simulink model "IntegratedFormationOptical"  (R2026a)
settings: Solver=ode4  StopTime=Tend  FixedStep=Ts
model workspace (MAT data in the model file):
  CASE = 3
  MODE = 2
  TACQ = 40
  TAUCPA = 0.005
  TX = [1; 1; 1; 2; 3]
  Tend = 50
  Ts = 0.001
  c0 = [0.824168944005; -0.579250814418; 0.824168944005; -0.579250814418; 0.824168944005; -0.579250814418; 0.676400226361; -0.507300169771; 0.44019405004; 0.711385027297]
  cfg.n = 4
  cfg.topology = 'mesh'
  cfg.seed = 101
  cfg.dt = 0.02
  cfg.T = 50
  cfg.J = 0.002
  cfg.b = 0.004
  cfg.tau = 0.08
  cfg.umax = 2e-06
  cfg.rateMax = 0.00012
  cfg.lambda = 8
  cfg.K = 8e-05
  cfg.phi = 8e-06
  cfg.kp = 64
  cfg.kd = 14
  cfg.ki = 8
  cfg.initialAngle = [2e-06; -1e-06]
  cfg.noise = 8e-08
  cfg.powerNoise = 0.008
  cfg.Pt = 0.5
  cfg.eta = 0.4
  cfg.divergence = 2e-05
  cfg.aperture = 0.1
  cfg.distance = 800000
  cfg.sensitivity = 1.5e-06
  cfg.capacity = 1000000000
  cfg.offered = 600000000
  cfg.packetBits = 12000
  cfg.c = 299792458
  cfg.processing = 0.0001
  cfg.method = 'proposed'
  cfg.controller = 'SMC'
  cfg.scenario = 'normal'
  cfg.faultStart = 42
  cfg.faultEnd = 48
  cfg.profile = 'sudden'
  cfg.severity = 1
  cfg.probeAmplitude = 6e-06
  cfg.probeDwell = 0.5
  cfg.maxCorrection = 3.5e-05
  cfg.detectRatio = 0.72
  cfg.decisionPeriod = 0.1
  cfg.warmup = 41
  cfg.edges = [1  2; 1  3; 1  4; 2  3; 3  4]
  cfg.m = 5
  cfg.version = '1.0.0'
  cfg.assumptions = 'Fixed sparse graph; one effective two-axis terminal per bidirectional edge; fluid single flow 1 to 2; no orbital propagation or atmospheric loss.'
  cfg.noiseSamples = [0.0535121228343 0.398971857605 -3.13116194418 0.785317147926 -0.646255228153 0.891855797063 0.932023533057 -1.5355153092 0.0745919923426 -0.661062844199 -0.294971205653 0.972557875124 ... (62625 elements, 2505x5x5)]
  distData = [0  0  0  0  0  0  0  0  0  0  0  0  0; 1  0  0  0  0  0  0  0  0  0  0  0  0; 2  0  0  0  0  0  0  0  0  0  0  0  0; 51  0  0  0  0  0  0  0  0  0  0  0  0]
  umax = 0.2
  x0 = [0.15; 0.22; -0.15; 0.15; -0.08; 0.12; 0.08; 0.18; -0.13; -0.14; 0.11; 0.13; -0.09; 0.12; 0.18; 0.16; 0.12; -0.07; 0.12; -0.13; 0.15; -0.13; -0.17; 0.12]
undefined symbols (not defined in the file or in its folder): terminal_parameters
settings Model: Creator=kaush  LastModifiedBy=kaush

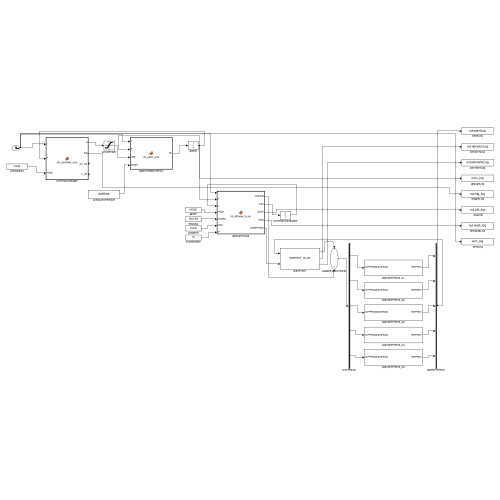
[thumbnail: Simulink's stored preview of the top-level diagram]
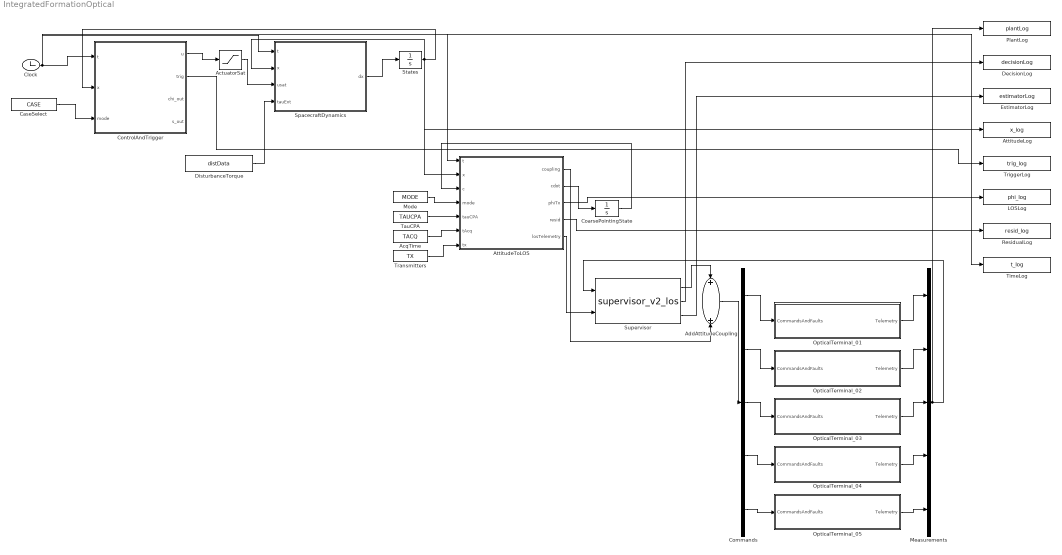
== system IntegratedFormationOptical ==
  AcqTime : Constant  Value=TACQ
  ActuatorSat : Saturate  UpperLimit=umax  LowerLimit=-umax
  AddAttitudeCoupling : Sum
  AttitudeLog : ToWorkspace  VariableName=x_log  SampleTime=cfg.dt
  AttitudeToLOS : MATLAB Function  TreatAsAtomicUnit=on
  CaseSelect : Constant  Value=CASE
  Clock : Clock
  CoarsePointingState : Integrator  InitialCondition=c0
  Commands : Demux  Outputs=[11 11 11 11 11]
  ControlAndTrigger : MATLAB Function  TreatAsAtomicUnit=on
  DecisionLog : ToWorkspace  VariableName=decisionLog  SaveFormat=Timeseries  SampleTime=-1
  DisturbanceTorque : FromWorkspace  VariableName=distData  Interpolate=off  OutputAfterFinalValue=Holding final value
  EstimatorLog : ToWorkspace  VariableName=estimatorLog  SaveFormat=Timeseries  SampleTime=-1
  LOSLog : ToWorkspace  VariableName=phi_log  SampleTime=cfg.dt
  Measurements : Mux  Inputs=5
  Mode : Constant  Value=MODE
  OpticalTerminal_01 : Subsystem
  OpticalTerminal_02 : Subsystem
  OpticalTerminal_03 : Subsystem
  OpticalTerminal_04 : Subsystem
  OpticalTerminal_05 : Subsystem
  PlantLog : ToWorkspace  VariableName=plantLog  SaveFormat=Timeseries  SampleTime=cfg.dt
  ResidualLog : ToWorkspace  VariableName=resid_log  SampleTime=cfg.dt
  SpacecraftDynamics : MATLAB Function  TreatAsAtomicUnit=on
  States : Integrator  InitialCondition=x0
  Supervisor : M-S-Function  FunctionName=supervisor_v2_los  Parameters=cfg
  TauCPA : Constant  Value=TAUCPA
  TimeLog : ToWorkspace  VariableName=t_log  SampleTime=cfg.dt
  Transmitters : Constant  Value=TX
  TriggerLog : ToWorkspace  VariableName=trig_log  SampleTime=Ts
  wires:
  Clock/1 -> ControlAndTrigger/1(t), SpacecraftDynamics/1(t), AttitudeToLOS/1(t), TimeLog/1
  States/1 -> ControlAndTrigger/2(x), SpacecraftDynamics/2(x), AttitudeToLOS/2(x), AttitudeLog/1
  CaseSelect/1 -> ControlAndTrigger/3(mode)
  ControlAndTrigger/1(u) -> ActuatorSat/1
  ActuatorSat/1 -> SpacecraftDynamics/3(usat)
  DisturbanceTorque/1 -> SpacecraftDynamics/4(tauExt)
  SpacecraftDynamics/1(dx) -> States/1
  CoarsePointingState/1 -> AttitudeToLOS/3(c)
  Mode/1 -> AttitudeToLOS/4(mode)
  TauCPA/1 -> AttitudeToLOS/5(tauCPA)
  AcqTime/1 -> AttitudeToLOS/6(tAcq)
  Transmitters/1 -> AttitudeToLOS/7(tx)
  AttitudeToLOS/2(cdot) -> CoarsePointingState/1
  Supervisor/1 -> AddAttitudeCoupling/1
  AttitudeToLOS/1(coupling) -> AddAttitudeCoupling/2
  AddAttitudeCoupling/1 -> Commands/1
  Commands/1 -> OpticalTerminal_01/1(CommandsAndFaults)
  OpticalTerminal_01/1(Telemetry) -> Measurements/1
  Commands/2 -> OpticalTerminal_02/1(CommandsAndFaults)
  OpticalTerminal_02/1(Telemetry) -> Measurements/2
  Commands/3 -> OpticalTerminal_03/1(CommandsAndFaults)
  OpticalTerminal_03/1(Telemetry) -> Measurements/3
  Commands/4 -> OpticalTerminal_04/1(CommandsAndFaults)
  OpticalTerminal_04/1(Telemetry) -> Measurements/4
  Commands/5 -> OpticalTerminal_05/1(CommandsAndFaults)
  OpticalTerminal_05/1(Telemetry) -> Measurements/5
  Measurements/1 -> Supervisor/1, PlantLog/1
  AttitudeToLOS/5(losTelemetry) -> Supervisor/2
  Supervisor/2 -> DecisionLog/1
  Supervisor/3 -> EstimatorLog/1
  ControlAndTrigger/2(trig) -> TriggerLog/1
  AttitudeToLOS/3(phiTx) -> LOSLog/1
  AttitudeToLOS/4(resid) -> ResidualLog/1

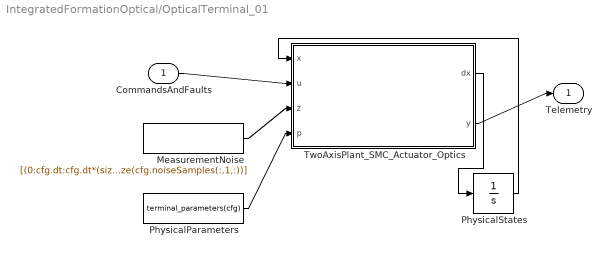
== system IntegratedFormationOptical/OpticalTerminal_01 ==
  CommandsAndFaults : Inport
  MeasurementNoise : FromWorkspace  VariableName=[(0:cfg.dt:cfg.dt*(size(cfg.noiseSamples,1)-1))' squeeze(cfg.noiseSamples(:,1,:))]  Interpolate=off  OutputAfterFinalValue=Holding final value
  PhysicalParameters : Constant  Value=terminal_parameters(cfg)
  PhysicalStates : Integrator  InitialCondition=[cfg.initialAngle;zeros(6,1)]
  TwoAxisPlant_SMC_Actuator_Optics : MATLAB Function  TreatAsAtomicUnit=on
  Telemetry : Outport
  wires:
  CommandsAndFaults/1 -> TwoAxisPlant_SMC_Actuator_Optics/2(u)
  PhysicalStates/1 -> TwoAxisPlant_SMC_Actuator_Optics/1(x)
  MeasurementNoise/1 -> TwoAxisPlant_SMC_Actuator_Optics/3(z)
  PhysicalParameters/1 -> TwoAxisPlant_SMC_Actuator_Optics/4(p)
  TwoAxisPlant_SMC_Actuator_Optics/1(dx) -> PhysicalStates/1
  TwoAxisPlant_SMC_Actuator_Optics/2(y) -> Telemetry/1

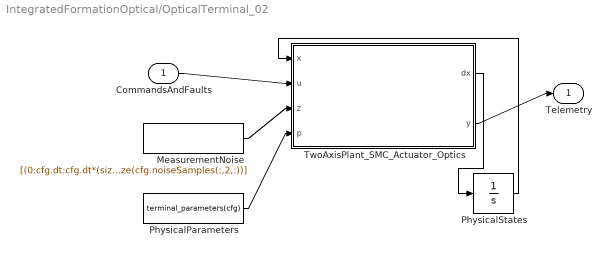
== system IntegratedFormationOptical/OpticalTerminal_02 ==
  CommandsAndFaults : Inport
  MeasurementNoise : FromWorkspace  VariableName=[(0:cfg.dt:cfg.dt*(size(cfg.noiseSamples,1)-1))' squeeze(cfg.noiseSamples(:,2,:))]  Interpolate=off  OutputAfterFinalValue=Holding final value
  PhysicalParameters : Constant  Value=terminal_parameters(cfg)
  PhysicalStates : Integrator  InitialCondition=[cfg.initialAngle;zeros(6,1)]
  TwoAxisPlant_SMC_Actuator_Optics : MATLAB Function  TreatAsAtomicUnit=on
  Telemetry : Outport
  wires:
  CommandsAndFaults/1 -> TwoAxisPlant_SMC_Actuator_Optics/2(u)
  PhysicalStates/1 -> TwoAxisPlant_SMC_Actuator_Optics/1(x)
  MeasurementNoise/1 -> TwoAxisPlant_SMC_Actuator_Optics/3(z)
  PhysicalParameters/1 -> TwoAxisPlant_SMC_Actuator_Optics/4(p)
  TwoAxisPlant_SMC_Actuator_Optics/1(dx) -> PhysicalStates/1
  TwoAxisPlant_SMC_Actuator_Optics/2(y) -> Telemetry/1

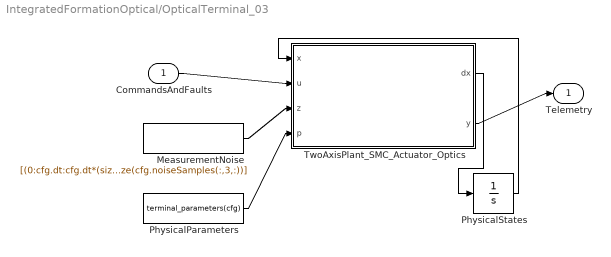
== system IntegratedFormationOptical/OpticalTerminal_03 ==
  CommandsAndFaults : Inport
  MeasurementNoise : FromWorkspace  VariableName=[(0:cfg.dt:cfg.dt*(size(cfg.noiseSamples,1)-1))' squeeze(cfg.noiseSamples(:,3,:))]  Interpolate=off  OutputAfterFinalValue=Holding final value
  PhysicalParameters : Constant  Value=terminal_parameters(cfg)
  PhysicalStates : Integrator  InitialCondition=[cfg.initialAngle;zeros(6,1)]
  TwoAxisPlant_SMC_Actuator_Optics : MATLAB Function  TreatAsAtomicUnit=on
  Telemetry : Outport
  wires:
  CommandsAndFaults/1 -> TwoAxisPlant_SMC_Actuator_Optics/2(u)
  PhysicalStates/1 -> TwoAxisPlant_SMC_Actuator_Optics/1(x)
  MeasurementNoise/1 -> TwoAxisPlant_SMC_Actuator_Optics/3(z)
  PhysicalParameters/1 -> TwoAxisPlant_SMC_Actuator_Optics/4(p)
  TwoAxisPlant_SMC_Actuator_Optics/1(dx) -> PhysicalStates/1
  TwoAxisPlant_SMC_Actuator_Optics/2(y) -> Telemetry/1

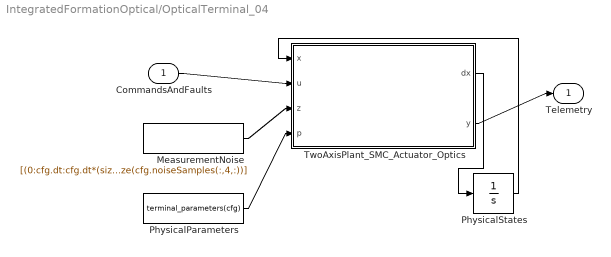
== system IntegratedFormationOptical/OpticalTerminal_04 ==
  CommandsAndFaults : Inport
  MeasurementNoise : FromWorkspace  VariableName=[(0:cfg.dt:cfg.dt*(size(cfg.noiseSamples,1)-1))' squeeze(cfg.noiseSamples(:,4,:))]  Interpolate=off  OutputAfterFinalValue=Holding final value
  PhysicalParameters : Constant  Value=terminal_parameters(cfg)
  PhysicalStates : Integrator  InitialCondition=[cfg.initialAngle;zeros(6,1)]
  TwoAxisPlant_SMC_Actuator_Optics : MATLAB Function  TreatAsAtomicUnit=on
  Telemetry : Outport
  wires:
  CommandsAndFaults/1 -> TwoAxisPlant_SMC_Actuator_Optics/2(u)
  PhysicalStates/1 -> TwoAxisPlant_SMC_Actuator_Optics/1(x)
  MeasurementNoise/1 -> TwoAxisPlant_SMC_Actuator_Optics/3(z)
  PhysicalParameters/1 -> TwoAxisPlant_SMC_Actuator_Optics/4(p)
  TwoAxisPlant_SMC_Actuator_Optics/1(dx) -> PhysicalStates/1
  TwoAxisPlant_SMC_Actuator_Optics/2(y) -> Telemetry/1

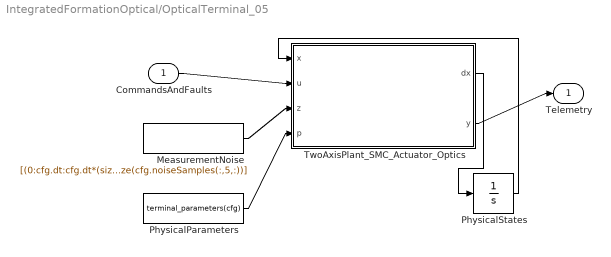
== system IntegratedFormationOptical/OpticalTerminal_05 ==
  CommandsAndFaults : Inport
  MeasurementNoise : FromWorkspace  VariableName=[(0:cfg.dt:cfg.dt*(size(cfg.noiseSamples,1)-1))' squeeze(cfg.noiseSamples(:,5,:))]  Interpolate=off  OutputAfterFinalValue=Holding final value
  PhysicalParameters : Constant  Value=terminal_parameters(cfg)
  PhysicalStates : Integrator  InitialCondition=[cfg.initialAngle;zeros(6,1)]
  TwoAxisPlant_SMC_Actuator_Optics : MATLAB Function  TreatAsAtomicUnit=on
  Telemetry : Outport
  wires:
  CommandsAndFaults/1 -> TwoAxisPlant_SMC_Actuator_Optics/2(u)
  PhysicalStates/1 -> TwoAxisPlant_SMC_Actuator_Optics/1(x)
  MeasurementNoise/1 -> TwoAxisPlant_SMC_Actuator_Optics/3(z)
  PhysicalParameters/1 -> TwoAxisPlant_SMC_Actuator_Optics/4(p)
  TwoAxisPlant_SMC_Actuator_Optics/1(dx) -> PhysicalStates/1
  TwoAxisPlant_SMC_Actuator_Optics/2(y) -> Telemetry/1

== matlab function IntegratedFormationOptical/OpticalTerminal_05/TwoAxisPlant_SMC_Actuator_Optics ==
  data: x input; dx output; u input; y output; z input; p input
function [dx,y]=terminal_kernel(x,u,z,p)
%#codegen
J=p(1);b=p(2);tau=p(3);umax=p(4);vmax=p(5);
theta=x(1:2);v=x(3:4);a=x(5:6);r=u(1:2);
ym=theta+u(7:8)+p(13)*u(11)*z(1:2);vm=v+p(13)*2*z(3:4);
e=ym-r;s=vm+p(6)*e;
if p(15)>0
 raw=J*(-p(9)*e-p(10)*vm-p(11)*x(7:8))+b*vm;
else
 raw=b*vm-J*p(6)*vm-J*p(7)*max(-1,min(1,s/p(8)));
end
cmd=max(-umax,min(umax,raw));
dv=(a-b*v)/J;
for k=1:2
 if abs(v(k))>=vmax && sign(v(k))*dv(k)>0,dv(k)=0;end
end
di=e;for k=1:2,if abs(raw(k))>umax,di(k)=0;end,end
dx=[max(-vmax,min(vmax,v));dv;(u(3)*cmd-a)/(tau*u(4));di];
err=theta+u(9:10);
power=p(12)*exp(-2*sum(err.^2)/p(16)^2)*max(0,u(5))*double(u(6)<=0);
q=power/p(17);pm=max(0,power*(1+p(14)*z(5)));
y=[r;theta;err;v;s;cmd;a;double(any(abs(raw)>umax));power;q;double(q>=1);ym;vm;pm;u(3);u(4);u(5)];
end

== matlab function IntegratedFormationOptical/SpacecraftDynamics ==
  data: t input; dx output; x input; usat input; tauExt input
function dx = int_plant_core(t, x, usat, tauExt)
%INT_PLANT_CORE  Project A spacecraft dynamics plus an optional external
%   disturbance torque, used only by the integrated model.
%   Calls the UNMODIFIED Project A plant sff_plant_core (eq. 1-2) and adds
%   J_i^-1 * tauExt_i to each spacecraft's angular acceleration.
%   tauExt : 12x1 [N*m], body frame, bypasses actuator effectiveness Gamma_i.
%#codegen
dx = sff_plant_core(t, x, usat);
Jd = [5.1 4.8 5.0
      4.9 4.9 5.1
      5.0 5.2 5.1
      4.8 5.1 4.9];            % same inertias as sff_params / sff_plant_core
for i = 1:4
    ks = 6*(i-1);
    dx(ks+4:ks+6) = dx(ks+4:ks+6) + tauExt(3*(i-1)+1:3*(i-1)+3) ./ Jd(i,:).';
end
end

== matlab function IntegratedFormationOptical/ControlAndTrigger ==
  settings: updateMethod=DISCRETE  sampleTime=Ts
  data: t input; u output; x input; mode input; trig output; chi_out output; s_out output
function [u, trig, chi_out, s_out] = sff_controller_core(t, x, mode)
%SFF_CONTROLLER_CORE  Distributed fault-tolerant attitude controller with
%   the three triggering mechanisms of Xie/Sheng/Chen (IEEE TAES 2024).
%
%   mode : 1 = Case 1, time-driven controller (31)
%          2 = Case 2, dynamic event-triggered controller (8)+(10)+(11)
%          3 = Case 3, self-triggered controller (8)+(26)
%
%   x = [sigma_1; omega_1; ... ; sigma_4; omega_4]

%#codegen

% ===================== Paper parameters ================================

A = [0 1 0 0
     1 0 1 0
     1 1 0 0
     1 0 0 0];

b = [1 0 0 0];

d = sum(A,2).' + b;

r     = 0.6;
k0    = 0.1;
alpha = 0.001 * ones(1,4);
delta = 0.3   * ones(1,4);
epsi  = 1e-4  * ones(1,4);
chi0  = 0.3   * ones(1,4);
beta1 = 5     * ones(1,4);
beta2 = 10    * ones(1,4);
gam   = 0.5   * ones(1,4);

% Theorem 1
k1 = 2*(gam.*beta1 + beta2) ./ d;
k2 = (k0 + 1) ./ (d .* delta);

% Inertia matrices
Jd = [5.1 4.8 5.0
      4.9 4.9 5.1
      5.0 5.2 5.1
      4.8 5.1 4.9];

% ||J_i^{-1}||_2 for diagonal inertia matrices
nJinv = 1 ./ min(Jd,[],2).';

n  = 4;
Ts = 1e-3;

% Case 1: 10 Hz
Tc1 = 0.1;


% ===================== Persistent trigger memory =======================

persistent isInit uHold sBcast oBcast skHold chi tNext

if isempty(isInit)

    isInit = true;

    % Initial commanded control
    uHold = zeros(12,1);

    % Initial broadcast states
    sBcast = zeros(12,1);
    oBcast = zeros(12,1);

    for j = 1:4

        kj = 6*(j-1);

        % Initial attitude
        sBcast(3*(j-1)+1 : 3*(j-1)+3) = ...
            x(kj+1 : kj+3);

        % Initial angular velocity
        oBcast(3*(j-1)+1 : 3*(j-1)+3) = ...
            x(kj+4 : kj+6);

    end

    % Sliding-variable memory
    skHold = zeros(12,1);

    % chi_i(0)
    chi = chi0(:);

    % Next scheduled trigger
    tNext = zeros(4,1);

end


% ===================== Reference trajectory =============================

[sd, od] = sff_ref_local(t);


% ===================== Snapshot of broadcast states =====================

sB = sBcast;
oB = oBcast;


% ===================== Outputs ==========================================

u     = uHold;
trig  = zeros(4,1);
s_out = zeros(12,1);


% ===================== Four spacecraft ================================

for i = 1:4

    ki = 3*(i-1);

    % Current spacecraft state
    sig = x(6*(i-1)+1 : 6*(i-1)+3);
    om  = x(6*(i-1)+4 : 6*(i-1)+6);


    % =================================================================
    % Formation errors
    % =================================================================

    e1 = b(i)*(sig - sd);
    e2 = b(i)*(om  - od);

    for j = 1:4

        if A(i,j) ~= 0

            e1 = e1 + ...
                (sig - sB(3*(j-1)+1 : 3*(j-1)+3));

            e2 = e2 + ...
                (om - oB(3*(j-1)+1 : 3*(j-1)+3));

        end

    end


    % =================================================================
    % Sliding variable
    % =================================================================

    s = e2 + r*e1;

    s_out(ki+1 : ki+3) = s;


    % =================================================================
    % CASE 1
    % Time-driven controller
    % =================================================================

    if mode == 1

        if t >= tNext(i) - Ts/2

            e1t = b(i)*(sig - sd);
            e2t = b(i)*(om  - od);

            for j = 1:4

                if A(i,j) ~= 0

                    e1t = e1t + ...
                        (sig - x(6*(j-1)+1 : 6*(j-1)+3));

                    e2t = e2t + ...
                        (om - x(6*(j-1)+4 : 6*(j-1)+6));

                end

            end

            st = e2t + r*e1t;

            Phi = 1 + norm(om) + norm(om)^2;

            u(ki+1 : ki+3) = ...
                -k1(i)*st ...
                -k2(i)*alpha(i)*Phi*sign(st);

            trig(i) = 1;

            tNext(i) = tNext(i) + Tc1;

        end


    % =================================================================
    % CASES 2 AND 3
    % =================================================================

    else

        % Equation (9)
        stil = ...
            skHold(ki+1 : ki+3) - s;

        nsk2 = ...
            skHold(ki+1 : ki+3).' * ...
            skHold(ki+1 : ki+3);

        fire = false;


        % =============================================================
        % CASE 2
        % Dynamic event-triggered controller
        % =============================================================

        if mode == 2

            if t <= 0

                fire = true;

            elseif (stil.'*stil - delta(i)*nsk2) ...
                    >= (chi(i) + epsi(i))

                fire = true;

            end


        % =============================================================
        % CASE 3
        % Self-triggered controller
        % =============================================================

        else

            if t >= tNext(i) - Ts/2

                fire = true;

            end

        end


        % =============================================================
        % Trigger event
        % =============================================================

        if fire

            % Broadcast current state
            sBcast(ki+1 : ki+3) = sig;
            oBcast(ki+1 : ki+3) = om;

            % Store current sliding variable
            skHold(ki+1 : ki+3) = s;

            % Equation (8)
            Phi = 1 + norm(om) + norm(om)^2;

            u(ki+1 : ki+3) = ...
                -k1(i)*s ...
                -k2(i)*alpha(i)*Phi*sign(s);

            trig(i) = 1;

            % Reset sampled error
            stil = zeros(3,1);

            nsk2 = s.'*s;


            % =========================================================
            % CASE 3
            % Self-trigger equation (26)
            % =========================================================

            if mode == 3

                ns = sqrt(nsk2);

                % -----------------------------------------------------
                % Equation (26)
                %
                % Factor 2 is included in the denominator.
                % -----------------------------------------------------

                den = 2*nJinv(i) * ...
                    ( ...
                    (n+1)*k1(i)*ns ...
                    + ((n+1)*k2(i) + 1)*alpha(i)*Phi ...
                    );


                % -----------------------------------------------------
                % Solve the implicit t_{k+1} expression using
                % fixed-point iteration.
                %
                % This implementation is compatible with the
                % MATLAB Function block / code generation.
                % -----------------------------------------------------

                tk1 = t;

                for it = 1:60

                    num = sqrt( ...
                        delta(i)*nsk2 ...
                        + chi0(i)* ...
                        exp(-(beta1(i)+beta2(i))*tk1) ...
                        + epsi(i) ...
                        );

                    tk1 = t + num/den;

                end


                % -----------------------------------------------------
                % Ensure the next trigger is at least one simulation
                % sample into the future.
                % -----------------------------------------------------

                if tk1 < t + Ts

                    tk1 = t + Ts;

                end

                tNext(i) = tk1;

            end

        end


        % =============================================================
        % Dynamic variable chi_i
        % =============================================================

        if mode == 2

            chid = ...
                -beta1(i)*chi(i) ...
                + beta2(i)*( ...
                    delta(i)*nsk2 ...
                    + epsi(i) ...
                    - stil.'*stil ...
                    );

            % Numerical integration
            chi(i) = chi(i) + Ts*chid;

        else

            % Self-triggered case
            chi(i) = ...
                chi0(i)* ...
                exp(-(beta1(i)+beta2(i))*t);

        end

    end

end


% ===================== Update persistent outputs ========================

uHold   = u;
chi_out = chi;

end


% ========================================================================
% Reference trajectory
% ========================================================================

function [sd, od] = sff_ref_local(t)
%#codegen

% Reference attitude
%
% sigma_d =
% [3 + 2sin(0.1t)
%  5 + 3cos(0.2t)
% -2 + cos(0.1t)] * 10^-3

sd = [ ...
     3 + 2*sin(0.1*t)
     5 + 3*cos(0.2*t)
    -2 + cos(0.1*t)] * 1e-3;


% Time derivative

sdd = [ ...
     0.2*cos(0.1*t)
    -0.6*sin(0.2*t)
    -0.1*sin(0.1*t)] * 1e-3;


% MRP kinematics:
%
% sigma_dot = G(sigma) omega
%
% omega_d = G(sigma_d)^(-1) sigma_dot_d

G = ...
    0.25*(1 - (sd.'*sd))*eye(3) ...
    + 0.5*sff_skew_local(sd) ...
    + 0.5*(sd*sd.');

od = G \ sdd;

end


% ========================================================================
% Skew-symmetric matrix
% ========================================================================

function S = sff_skew_local(v)
%#codegen

S = [ ...
       0   -v(3)   v(2)
     v(3)     0  -v(1)
    -v(2)   v(1)     0
    ];

end

== matlab function IntegratedFormationOptical/AttitudeToLOS ==
  data: t input; coupling output; x input; c input; mode input; tauCPA input; tAcq input; tx input; cdot output; phiTx output; resid output; losTelemetry output
function [coupling, cdot, phiTx, resid, losTelemetry] = int_attitude_to_los(t, x, c, mode, tauCPA, tAcq, tx)
%INT_ATTITUDE_TO_LOS  The single interface between Project A and Project B.
%
%   Spacecraft attitude error -> optical line-of-sight (LOS) error of the
%   terminal on each optical link.
%
%   x      : 24x1 Project A state [sigma_1; omega_1; ...; sigma_4; omega_4]
%   c      : 2m x1 coarse-pointing (CPA) compensation state [rad]
%   mode   : 0 = uncoupled (baselines)
%            1 = raw coupling, no coarse pointing
%            2 = CPA compensation; the fine terminal and supervisor are NOT told
%                about the residual (it acts as an unknown optical offset)
%            3 = CPA compensation + the measurable CPA residual d is given to
%                the Project B supervisor as telemetry, used only in its optical
%                power model (supervisor_v2_los). Fine-stage commands unchanged.
%   tAcq   : link acquisition time; coupling active for t >= tAcq
%   tx     : m x1 transmitting spacecraft of each link
%
%   Equations (small angles, transmitting spacecraft i):
%     sigma_e  = sigma_i - sigma_d(t)                                   (Project A error)
%     phi      = 4*atan(|sigma_e|) * sigma_e/|sigma_e|                  (MRP -> rotation vector)
%     phi_LOS  = [phi_y; phi_z]                                         (boresight along body +x)
%     CPA:       c_dot = (phi_LOS - c)/tauCPA,   d = phi_LOS - c
%     Plant:     optical error = theta_terminal + offset_fault + d       -> u(9:10) += d
%     Mode 3:    losTelemetry = d  (supervisor predicts P = P0*g*exp(-2|q+d+delta|^2/alpha^2))
%   No fault label, fault schedule or fault parameter is used here.
%#codegen
m = numel(tx);
coupling = zeros(11*m, 1);
losTelemetry = zeros(2*m, 1);
cdot  = zeros(2*m, 1);
phiTx = zeros(2*m, 1);
resid = zeros(2*m, 1);

sd = [ 3 + 2*sin(0.1*t)
       5 + 3*cos(0.2*t)
      -2 +   cos(0.1*t)] * 1e-3;                   % Project A reference sigma_d(t)

for j = 1:m
    i  = tx(j);
    se = x(6*(i-1)+1 : 6*(i-1)+3) - sd;
    ns = norm(se);
    if ns > 0
        phi = 4*atan(ns) * se / ns;
    else
        phi = zeros(3,1);
    end
    p  = phi(2:3);
    k  = 2*j-1:2*j;
    phiTx(k) = p;
    cdot(k)  = (p - c(k)) / tauCPA;
    if mode == 1
        d = p;
    elseif mode >= 2
        d = p - c(k);
    else
        d = zeros(2,1);
    end
    if t < tAcq
        d = zeros(2,1);
    end
    resid(k) = d;
    coupling(11*(j-1)+9 : 11*(j-1)+10) = d;              % physics: LOS disturbance
    if mode == 3
        losTelemetry(k) = d;                              % known to the spacecraft
    end
end
end

== matlab function IntegratedFormationOptical/OpticalTerminal_01/TwoAxisPlant_SMC_Actuator_Optics ==
  data: x input; dx output; u input; y output; z input; p input
function [dx,y]=terminal_kernel(x,u,z,p)
%#codegen
J=p(1);b=p(2);tau=p(3);umax=p(4);vmax=p(5);
theta=x(1:2);v=x(3:4);a=x(5:6);r=u(1:2);
ym=theta+u(7:8)+p(13)*u(11)*z(1:2);vm=v+p(13)*2*z(3:4);
e=ym-r;s=vm+p(6)*e;
if p(15)>0
 raw=J*(-p(9)*e-p(10)*vm-p(11)*x(7:8))+b*vm;
else
 raw=b*vm-J*p(6)*vm-J*p(7)*max(-1,min(1,s/p(8)));
end
cmd=max(-umax,min(umax,raw));
dv=(a-b*v)/J;
for k=1:2
 if abs(v(k))>=vmax && sign(v(k))*dv(k)>0,dv(k)=0;end
end
di=e;for k=1:2,if abs(raw(k))>umax,di(k)=0;end,end
dx=[max(-vmax,min(vmax,v));dv;(u(3)*cmd-a)/(tau*u(4));di];
err=theta+u(9:10);
power=p(12)*exp(-2*sum(err.^2)/p(16)^2)*max(0,u(5))*double(u(6)<=0);
q=power/p(17);pm=max(0,power*(1+p(14)*z(5)));
y=[r;theta;err;v;s;cmd;a;double(any(abs(raw)>umax));power;q;double(q>=1);ym;vm;pm;u(3);u(4);u(5)];
end

== matlab function IntegratedFormationOptical/OpticalTerminal_02/TwoAxisPlant_SMC_Actuator_Optics ==
  data: x input; dx output; u input; y output; z input; p input
function [dx,y]=terminal_kernel(x,u,z,p)
%#codegen
J=p(1);b=p(2);tau=p(3);umax=p(4);vmax=p(5);
theta=x(1:2);v=x(3:4);a=x(5:6);r=u(1:2);
ym=theta+u(7:8)+p(13)*u(11)*z(1:2);vm=v+p(13)*2*z(3:4);
e=ym-r;s=vm+p(6)*e;
if p(15)>0
 raw=J*(-p(9)*e-p(10)*vm-p(11)*x(7:8))+b*vm;
else
 raw=b*vm-J*p(6)*vm-J*p(7)*max(-1,min(1,s/p(8)));
end
cmd=max(-umax,min(umax,raw));
dv=(a-b*v)/J;
for k=1:2
 if abs(v(k))>=vmax && sign(v(k))*dv(k)>0,dv(k)=0;end
end
di=e;for k=1:2,if abs(raw(k))>umax,di(k)=0;end,end
dx=[max(-vmax,min(vmax,v));dv;(u(3)*cmd-a)/(tau*u(4));di];
err=theta+u(9:10);
power=p(12)*exp(-2*sum(err.^2)/p(16)^2)*max(0,u(5))*double(u(6)<=0);
q=power/p(17);pm=max(0,power*(1+p(14)*z(5)));
y=[r;theta;err;v;s;cmd;a;double(any(abs(raw)>umax));power;q;double(q>=1);ym;vm;pm;u(3);u(4);u(5)];
end

== matlab function IntegratedFormationOptical/OpticalTerminal_03/TwoAxisPlant_SMC_Actuator_Optics ==
  data: x input; dx output; u input; y output; z input; p input
function [dx,y]=terminal_kernel(x,u,z,p)
%#codegen
J=p(1);b=p(2);tau=p(3);umax=p(4);vmax=p(5);
theta=x(1:2);v=x(3:4);a=x(5:6);r=u(1:2);
ym=theta+u(7:8)+p(13)*u(11)*z(1:2);vm=v+p(13)*2*z(3:4);
e=ym-r;s=vm+p(6)*e;
if p(15)>0
 raw=J*(-p(9)*e-p(10)*vm-p(11)*x(7:8))+b*vm;
else
 raw=b*vm-J*p(6)*vm-J*p(7)*max(-1,min(1,s/p(8)));
end
cmd=max(-umax,min(umax,raw));
dv=(a-b*v)/J;
for k=1:2
 if abs(v(k))>=vmax && sign(v(k))*dv(k)>0,dv(k)=0;end
end
di=e;for k=1:2,if abs(raw(k))>umax,di(k)=0;end,end
dx=[max(-vmax,min(vmax,v));dv;(u(3)*cmd-a)/(tau*u(4));di];
err=theta+u(9:10);
power=p(12)*exp(-2*sum(err.^2)/p(16)^2)*max(0,u(5))*double(u(6)<=0);
q=power/p(17);pm=max(0,power*(1+p(14)*z(5)));
y=[r;theta;err;v;s;cmd;a;double(any(abs(raw)>umax));power;q;double(q>=1);ym;vm;pm;u(3);u(4);u(5)];
end

== matlab function IntegratedFormationOptical/OpticalTerminal_04/TwoAxisPlant_SMC_Actuator_Optics ==
  data: x input; dx output; u input; y output; z input; p input
function [dx,y]=terminal_kernel(x,u,z,p)
%#codegen
J=p(1);b=p(2);tau=p(3);umax=p(4);vmax=p(5);
theta=x(1:2);v=x(3:4);a=x(5:6);r=u(1:2);
ym=theta+u(7:8)+p(13)*u(11)*z(1:2);vm=v+p(13)*2*z(3:4);
e=ym-r;s=vm+p(6)*e;
if p(15)>0
 raw=J*(-p(9)*e-p(10)*vm-p(11)*x(7:8))+b*vm;
else
 raw=b*vm-J*p(6)*vm-J*p(7)*max(-1,min(1,s/p(8)));
end
cmd=max(-umax,min(umax,raw));
dv=(a-b*v)/J;
for k=1:2
 if abs(v(k))>=vmax && sign(v(k))*dv(k)>0,dv(k)=0;end
end
di=e;for k=1:2,if abs(raw(k))>umax,di(k)=0;end,end
dx=[max(-vmax,min(vmax,v));dv;(u(3)*cmd-a)/(tau*u(4));di];
err=theta+u(9:10);
power=p(12)*exp(-2*sum(err.^2)/p(16)^2)*max(0,u(5))*double(u(6)<=0);
q=power/p(17);pm=max(0,power*(1+p(14)*z(5)));
y=[r;theta;err;v;s;cmd;a;double(any(abs(raw)>umax));power;q;double(q>=1);ym;vm;pm;u(3);u(4);u(5)];
end
